simulink model "Jacobiano"  (R2026b)
settings: Solver=VariableStepAuto  StopTime=5
libraries: simulink_extras x8
settings Model: Creator=Usuario  LastModifiedBy=Usuario

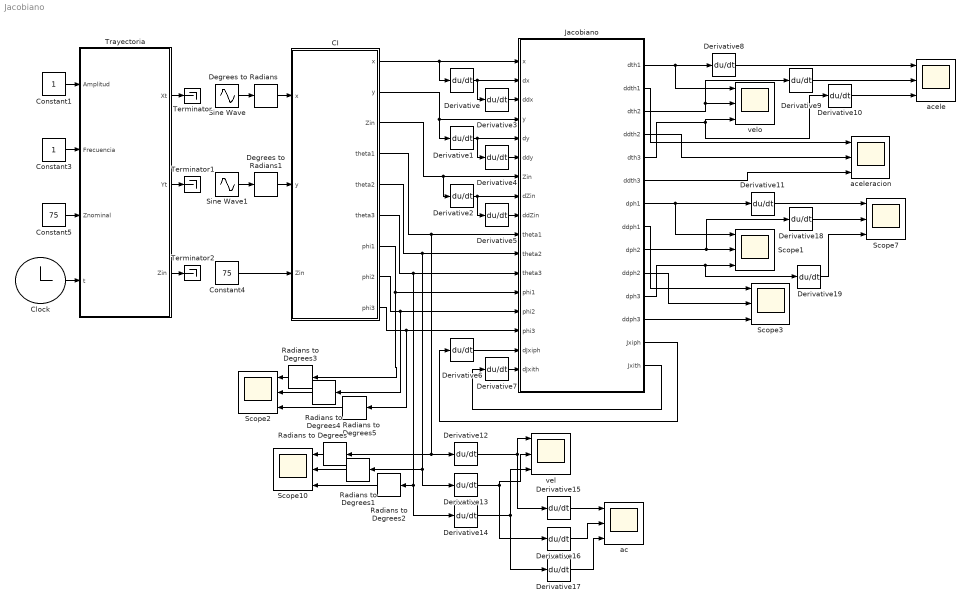
== system Jacobiano ==
  CI : MATLAB Function  TreatAsAtomicUnit=on
  Clock : Clock
  Constant1 : Constant
  Constant3 : Constant
  Constant4 : Constant  Value=75
  Constant5 : Constant  Value=75
  Degrees to Radians : simulink_extras/Transformations/Degrees to Radians
  Degrees to Radians1 : simulink_extras/Transformations/Degrees to Radians
  Derivative{,1..19} (20 alike) : Derivative
  Jacobiano : MATLAB Function  TreatAsAtomicUnit=on
  Radians to Degrees{,1..5} (6 alike) : simulink_extras/Transformations/Radians to Degrees
  Scope{1..3,7,10} (5 alike) : Scope  NumInputPorts=3
      Scope1 settings: ActiveDisplayYMinimum=-1  ActiveDisplayYMaximum=1
      Scope10 settings: ActiveDisplayYMinimum=-20.813147785255723  ActiveDisplayYMaximum=-7.1302672970198175  DataLoggingVariableName=ScopeData9
      Scope2 settings: ActiveDisplayYMinimum=-60.013633524403545  ActiveDisplayYMaximum=-57.700290830793769  DataLoggingVariableName=ScopeData6
      Scope3 settings: ActiveDisplayYMinimum=-0.85432884530891662  ActiveDisplayYMaximum=0.83684422936137559  DataLoggingVariableName=ScopeData2
      Scope7 settings: ActiveDisplayYMinimum=-17.205642787025777  ActiveDisplayYMaximum=17.09496293081693  DataLoggingVariableName=ScopeData5
  Sine Wave : Sin  Amplitude=5  SampleTime=0
  Sine Wave1 : Sin  Amplitude=5  Phase=pi/2  SampleTime=0
  Terminator : Terminator
  Terminator1 : Terminator
  Terminator2 : Terminator
  Trayectoria : MATLAB Function  TreatAsAtomicUnit=on
  ac : Scope  NumInputPorts=3
      settings: ActiveDisplayYMinimum=-1.0495453900450091  ActiveDisplayYMaximum=1.0934338180517422  DataLoggingVariableName=ScopeData8
  acele : Scope  NumInputPorts=3
      settings: ActiveDisplayYMinimum=-1.0318431328068014  ActiveDisplayYMaximum=1.110984928339434  DataLoggingVariableName=ScopeData3
  aceleracion : Scope  NumInputPorts=3
      settings: ActiveDisplayYMinimum=-1.0301694874355052  ActiveDisplayYMaximum=1.1121564633477239
  vel : Scope  NumInputPorts=3
      settings: ActiveDisplayYMinimum=-0.11999611177199715  ActiveDisplayYMaximum=0.11998383452322441  DataLoggingVariableName=ScopeData7
  velo : Scope  NumInputPorts=3
      settings: ActiveDisplayYMinimum=-0.1188290465740519  ActiveDisplayYMaximum=0.12436919945967165  DataLoggingVariableName=ScopeData4
  wires:
  Constant1/1 -> Trayectoria/1(Amplitud)
  Constant3/1 -> Trayectoria/2(Frecuencia)
  Constant5/1 -> Trayectoria/3(Znominal)
  Clock/1 -> Trayectoria/4(t)
  CI/2(y) -> Derivative1/1, Jacobiano/4(y)
  CI/3(Zin) -> Derivative2/1, Jacobiano/7(Zin)
  CI/4(theta1) -> Jacobiano/10(theta1), Derivative12/1, Radians to Degrees/1
  CI/5(theta2) -> Derivative13/1, Radians to Degrees1/1, Jacobiano/11(theta2)
  CI/6(theta3) -> Radians to Degrees2/1, Derivative14/1, Jacobiano/12(theta3)
  CI/9(phi3) -> Radians to Degrees5/1, Jacobiano/15(phi3)
  Derivative/1 -> Derivative3/1, Jacobiano/2(dx)
  Derivative1/1 -> Derivative4/1, Jacobiano/5(dy)
  Derivative2/1 -> Derivative5/1, Jacobiano/8(dZin)
  Jacobiano/3(dth2) -> Derivative9/1, velo/2
  Jacobiano/9(dph2) -> Derivative18/1, Scope1/2
  Jacobiano/7(dph1) -> Derivative11/1, Scope1/1
  Jacobiano/11(dph3) -> Derivative19/1, Scope1/3
  Jacobiano/5(dth3) -> Derivative10/1, velo/3
  Jacobiano/1(dth1) -> Derivative8/1, velo/1
  CI/1(x) -> Derivative/1, Jacobiano/1(x)
  Derivative3/1 -> Jacobiano/3(ddx)
  Derivative4/1 -> Jacobiano/6(ddy)
  Derivative5/1 -> Jacobiano/9(ddZin)
  Derivative6/1 -> Jacobiano/16(dJxiph)
  Derivative7/1 -> Jacobiano/17(dJxith)
  Jacobiano/13(Jxiph) -> Derivative6/1
  Jacobiano/14(Jxith) -> Derivative7/1
  Jacobiano/6(ddth3) -> aceleracion/3
  Jacobiano/4(ddth2) -> aceleracion/2
  Jacobiano/2(ddth1) -> aceleracion/1
  Jacobiano/12(ddph3) -> Scope3/3
  Jacobiano/10(ddph2) -> Scope3/2
  Jacobiano/8(ddph1) -> Scope3/1
  Derivative8/1 -> acele/1
  Derivative10/1 -> acele/3
  Derivative9/1 -> acele/2
  Derivative11/1 -> Scope7/1
  Derivative13/1 -> Derivative16/1, vel/2
  Derivative12/1 -> Derivative15/1, vel/1
  Derivative14/1 -> Derivative17/1, vel/3
  Derivative15/1 -> ac/1
  Derivative16/1 -> ac/2
  Derivative17/1 -> ac/3
  Radians to Degrees/1 -> Scope10/1
  Radians to Degrees1/1 -> Scope10/2
  Radians to Degrees2/1 -> Scope10/3
  Derivative18/1 -> Scope7/2
  Derivative19/1 -> Scope7/3
  Trayectoria/1(Xt) -> Terminator/1
  Trayectoria/2(Yt) -> Terminator1/1
  Trayectoria/3(Zin) -> Terminator2/1
  Sine Wave/1 -> Degrees to Radians/1
  Sine Wave1/1 -> Degrees to Radians1/1
  Degrees to Radians/1 -> CI/1("x ")
  Degrees to Radians1/1 -> CI/2("y ")
  Constant4/1 -> CI/3("Zin ")
  Radians to Degrees5/1 -> Scope2/3
  Radians to Degrees4/1 -> Scope2/2
  Radians to Degrees3/1 -> Scope2/1
  CI/8(phi2) -> Radians to Degrees4/1, Jacobiano/14(phi2)
  CI/7(phi1) -> Radians to Degrees3/1, Jacobiano/13(phi1)

== matlab function Jacobiano/Jacobiano ==
  data: x input; dx input; ddx input; dth1 output; ddth1 output; y input; dy input; ddy input; Zin input; dZin input; ddZin input; dth2 output; ddth2 output; theta1 input; theta2 input; theta3 input; phi1 input; phi2 input; phi3 input; dJxiph input; dth3 output; ddth3 output; dph1 output; ddph1 output; dph2 output; ddph2 output; dph3 output; ddph3 output; Jxiph output; Jxith output; dJxith input
function [dth1,ddth1, dth2,ddth2, dth3,ddth3, dph1,ddph1, dph2,ddph2, dph3,ddph3, Jxiph, Jxith] = fcn(x,dx,ddx,y,dy,ddy,Zin,dZin,ddZin,theta1, theta2, theta3, phi1, phi2, phi3,dJxiph,dJxith)
%% Constantes
p  = 55;
b  = 50;
l1 = 45;
l2 = 75;
Ax = x;
Ay = y;
f1 = (-sin(Ax)*sin(Ay))/(cos(Ax)+cos(Ay));
Az = atan(f1);
alfa1 = deg2rad(0);
alfa2 = deg2rad(120);
alfa3 = deg2rad(240);
Oz = Zin;

R = [ cos(Ay)*cos(Az)                          -cos(Ay)*sin(Az)                          sin(Ay)
      cos(Ax)*sin(Az)+cos(Az)*sin(Ax)*sin(Ay)    cos(Ax)*cos(Az)-sin(Ax)*sin(Ay)*sin(Az)  -cos(Ay)*sin(Ax)
      sin(Ax)*sin(Az)-cos(Ax)*cos(Az)*sin(Ay)    cos(Az)*sin(Ax)+cos(Ax)*sin(Ay)*sin(Az)   cos(Ax)*cos(Ay)];

Rz1 = [cos(alfa1) -sin(alfa1) 0; sin(alfa1) cos(alfa1) 0; 0 0 1];
Rz2 = [cos(alfa2) -sin(alfa2) 0; sin(alfa2) cos(alfa2) 0; 0 0 1];
Rz3 = [cos(alfa3) -sin(alfa3) 0; sin(alfa3) cos(alfa3) 0; 0 0 1];

P = [p; 0; 0];
ux = R(1,1); 
uy = R(1,2); 
vy = R(2,2);
Ox = (p*(ux-vy))/2;
Oy = -uy*p;
T  = [Ox; Oy; Oz];

O1 = T + (R*Rz1*P);
O2 = T + (R*Rz2*P);
O3 = T + (R*Rz3*P);

th1 = theta1; 
th2 = theta2; 
th3 = theta3;

%% Jacobiano de la restricción de cada pierna (lD, E)
lD1 = [-2*cos(alfa1)*(b+l1*cos(th1))+2*O1(1)   0   2*cos(alfa1)^2*(O1(3)+l1*sin(th1))];
E1  =  2*l1*cos(alfa1)*(cos(alfa1)*cos(th1)*O1(3) + (-b*cos(alfa1)+O1(1))*sin(th1));

lD2 = [-2*cos(alfa2)*(b+l1*cos(th2))+2*O2(1)   0   2*cos(alfa2)^2*(O2(3)+l1*sin(th2))];
E2  =  2*l1*cos(alfa2)*(cos(alfa2)*cos(th2)*O2(3) + (-b*cos(alfa2)+O2(1))*sin(th2));

lD3 = [-2*cos(alfa3)*(b+l1*cos(th3))+2*O3(1)   0   2*cos(alfa3)^2*(O3(3)+l1*sin(th3))];
E3  =  2*l1*cos(alfa3)*(cos(alfa3)*cos(th3)*O3(3) + (-b*cos(alfa3)+O3(1))*sin(th3));

Js = [lD1  0  0  0  0  0  0
       0   0  0 lD2 0  0  0
       0   0  0  0  0  0 lD3];

Jth = [E1  0  0
        0  E2 0
        0  0  E3];
dlX=[dZin; dx; dy];

%% Jacobiano de orientación pierna<-plataforma 
Jto1 = [1 0 0                    0                                           (-p*sin(Ay)*cos(alfa1+Az))              (-p*cos(Ay)*sin(alfa1+Az))
        0 1 0 p*((cos(Ax)*sin(Ay)*cos(alfa1+Az))-sin(Ax)*sin(alfa1+Az))  (p*sin(Ax)*cos(Ay)*cos(alfa1+Az))  p*(cos(Ax)*cos(alfa1+Az)-(sin(Ax)*sin(Ay)*sin(alfa1+Az)))
        0 0 1 p*((sin(Ax)*sin(Ay)*cos(alfa1+Az))+cos(Ax)*sin(alfa1+Az)) (-p*cos(Ax)*cos(Ay)*cos(alfa1+Az))  p*(sin(Ax)*cos(alfa1+Az)+(cos(Ax)*sin(Ay)*sin(alfa1+Az)))];

Jto2 = [1 0 0                    0                                           (-p*sin(Ay)*cos(alfa2+Az))              (-p*cos(Ay)*sin(alfa2+Az))
        0 1 0 p*((cos(Ax)*sin(Ay)*cos(alfa2+Az))-sin(Ax)*sin(alfa2+Az))  (p*sin(Ax)*cos(Ay)*cos(alfa2+Az))  p*(cos(Ax)*cos(alfa2+Az)-(sin(Ax)*sin(Ay)*sin(alfa2+Az)))
        0 0 1 p*((sin(Ax)*sin(Ay)*cos(alfa2+Az))+cos(Ax)*sin(alfa2+Az)) (-p*cos(Ax)*cos(Ay)*cos(alfa2+Az))  p*(sin(Ax)*cos(alfa2+Az)+(cos(Ax)*sin(Ay)*sin(alfa2+Az)))];

Jto3 = [1 0 0                    0                                           (-p*sin(Ay)*cos(alfa3+Az))              (-p*cos(Ay)*sin(alfa3+Az))
        0 1 0 p*((cos(Ax)*sin(Ay)*cos(alfa3+Az))-sin(Ax)*sin(alfa3+Az))  (p*sin(Ax)*cos(Ay)*cos(alfa3+Az))  p*(cos(Ax)*cos(alfa3+Az)-(sin(Ax)*sin(Ay)*sin(alfa3+Az)))
        0 0 1 p*((sin(Ax)*sin(Ay)*cos(alfa3+Az))+cos(Ax)*sin(alfa3+Az)) (-p*cos(Ax)*cos(Ay)*cos(alfa3+Az))  p*(sin(Ax)*cos(alfa3+Az)+(cos(Ax)*sin(Ay)*sin(alfa3+Az)))];

Jts = [Jto1; Jto2; Jto3];

%% Jacobiano de la tarea independiente (x,y -> [Ax,Ay,Az])
Jox = [0 -(p*cos(Ay)*sin(Ay)*(cos(Ax)+cos(Ay)*sin(Ax)*sin(Ay)))/(2*(1+cos(Ax)*cos(Ay))^2) ...
         -(p*cos(Ay)*sin(Ax)*(cos(Ax)+cos(Ay)+sin(Ax)*sin(Ay)))/(2*(1+cos(Ax)*cos(Ay))^2)];
Joy = [0 -(p*cos(Ay)*sin(Ay)*(cos(Ax)+cos(Ay)))/((1+cos(Ax)*cos(Ay))^2) ...
         -(p*sin(Ax)*(sin(Ax)^2*sin(Ay)^2-cos(Ay)^4-cos(Ax)^2*cos(Ay)^2-1/4*cos(Ax)*(5*cos(Ay)+3*cos(Ay)^3)))/((1+cos(Ax)*cos(Ay))^3)];
JAz = [0 -sin(Ay)/(1+cos(Ax)*cos(Ay))  -sin(Ax)/(1+cos(Ax)*cos(Ay))];
I3x3 = eye(3);

Jxit = [Jox; Joy; I3x3; JAz];
Jxith = (-inv(Jth))*Js*Jts*Jxit; 
dlth=Jxith*dlX;
dth1=dlth(1);
dth2=dlth(2);
dth3=dlth(3);

JSph1 = [0 0 -1/l2*cos(phi1)];
Jth1ph1 = -l1*cos(th1)/l2*cos(phi1);
JSph2 = [0 0 -1/l2*cos(phi2)];
Jth2ph2 = -l1*cos(th2)/l2*cos(phi2);
JSph3 = [0 0 -1/l2*cos(phi3)];
Jth3ph3 = -l1*cos(th3)/l2*cos(phi3);

JSph = [JSph1 0 0   0   0 0   0
          0   0 0 JSph2 0 0   0
          0   0 0   0   0 0 JSph3];
Jthph = [Jth1ph1    0        0
            0    Jth2ph2     0
            0       0    Jth3ph3];

Jxis  = Jts*Jxit;
Jxiph = (JSph*Jxis + Jthph*Jxith);   
dlph=Jxiph*dlX;
dph1=dlph(1);
dph2=dlph(2);
dph3=dlph(3);
%%segunda derivada
ddlX=[ddZin;ddx;ddy];
ddlth=dJxith*dlX+Jxith*ddlX;
ddth1=ddlth(1);
ddth2=ddlth(2);
ddth3=ddlth(3);

ddlph=dJxiph*dlX+Jxiph*ddlX;
ddph1=ddlph(1);
ddph2=ddlph(2);
ddph3=ddlph(3);
end

== matlab function Jacobiano/Trayectoria ==
  data: Amplitud input; Xt output; Frecuencia input; Znominal input; Yt output; Zin output; t input
function [Xt,Yt,Zin] = fcn(Amplitud, Frecuencia, Znominal, t)
A_deg      = Amplitud;      
f_hz       = Frecuencia;    
Zin_nom    = Znominal;    
sentido    = 1;      % +1 = antihorario, -1 = horario
w = 2*pi*f_hz;

Xt =2* A_deg * cos(w*t);
Yt =2* sentido * A_deg * sin(w*t);
Zin = Zin_nom;
end

== matlab function Jacobiano/CI ==
  data: x output; y output; Zin output; x input; theta1 output; y input; Zin input; theta2 output; theta3 output; phi1 output; phi2 output; phi3 output
function [x,y,Zin,theta1, theta2, theta3, phi1, phi2,phi3] = fcn(x,y, Zin)
%%constantes
p  = 55;   
b  = 50;    
l1 = 45;   
l2 = 75;  
%% ============================================================
Ax = x;
Ay = y;
f1=(-sin(Ax)*sin(Ay))/(cos(Ax)+cos(Ay));
Az=atan(f1);
alfa1 = deg2rad(0);
alfa2 = deg2rad(120);
alfa3 = deg2rad(240);
Oz = Zin;

R = [ cos(Ay)*cos(Az)                          -cos(Ay)*sin(Az)                          sin(Ay)
      cos(Ax)*sin(Az)+cos(Az)*sin(Ax)*sin(Ay)    cos(Ax)*cos(Az)-sin(Ax)*sin(Ay)*sin(Az)  -cos(Ay)*sin(Ax)
      sin(Ax)*sin(Az)-cos(Ax)*cos(Az)*sin(Ay)    cos(Az)*sin(Ax)+cos(Ax)*sin(Ay)*sin(Az)   cos(Ax)*cos(Ay)];
Rz1 = [cos(alfa1) -sin(alfa1) 0; sin(alfa1) cos(alfa1) 0; 0 0 1];
Rz2 = [cos(alfa2) -sin(alfa2) 0; sin(alfa2) cos(alfa2) 0; 0 0 1];
Rz3 = [cos(alfa3) -sin(alfa3) 0; sin(alfa3) cos(alfa3) 0; 0 0 1];
P = [p; 0; 0];
ux = R(1,1); uy = R(1,2); vy = R(2,2);
Ox = (p*(ux-vy))/2;
Oy = -uy*p;
T  = [Ox, Oy, Oz];
O1 = T' + (R*Rz1*P);
O2 = T' + (R*Rz2*P);
O3 = T' + (R*Rz3*P);

%% ============================================================
    function [th,phi] = solveLeg(O, alfa, b, l1, l2)
    A = 2*l1*cos(alfa)*(b*cos(alfa) - O(1));
    B = 2*l1*O(3)*cos(alfa)^2;
    C = O(1)^2 - 2*b*O(1)*cos(alfa) + cos(alfa)^2*(b^2 + l1^2 - l2^2 + O(3)^2);

    %disc = A^2 + B^2 - C^2;   % si es negativo -> pose inalcanzable
    f_sol1 =(-B+sqrt(A^2+B^2-C^2))\(C-A);
    % f_sol2 = (C - A) / (-B - sqrt(disc)); 

    Ang1 = 2*atan(f_sol1);
    th = (-Ang1)-pi; 

    Cphi11=(O(1)-cos(alfa)*(b+l1*cos(Ang1+pi)))/(l2*cos(alfa));
    Sphi11=(-O(3)+l1*sin(Ang1+pi))/l2;

    phi=(atan2(Cphi11,Sphi11))+pi/2;
    end
[theta1,phi1] = solveLeg(O1, alfa1, b, l1, l2);
[theta2,phi2] = solveLeg(O2, alfa2, b, l1, l2);
[theta3,phi3] = solveLeg(O3, alfa3, b, l1, l2);

end
